simulink model "Model_31_02_2"  (R2024b)
settings: Solver=FixedStepAuto  StartTime=0.0  StopTime=20  FixedStep=0.01  RelTol=1e-3
values from neighbouring files (symbols this model uses):
  b = pend1.b    [InversePODE.m]    (also in Laboratorio_2_Pendolo_inverso_struct.m = 0.001; TESTTT.m = 13.516; errori.m = 0.001; state_space1.m)
  c = pend1.c    [InversePODE.m]    (also in Laboratorio_2_Pendolo_inverso_struct.m = 0.1; TESTTT.m = 0.1; errori.m = 0.1; state_space1.m)
  F = -pend1.Kp*x_n_l_NL(:,3) - pend1.Kd * x_n_l_NL(:,4)    [Laboratorio_2_Pendolo_inverso_struct.m]    (also in TESTTT.m = -Kp*x_n_l_NL(:,3) - Kd * x_n_l_NL(:,4))
  g = pend1.g    [InversePODE.m]    (also in InversePODE_RNL.m; Laboratorio_2_Pendolo_inverso_struct.m = 9.81; TESTTT.m = 9.81; errori.m = 9.81)
  l = pend1.l    [InversePODE.m]    (also in InversePODE_RNL.m; Laboratorio_2_Pendolo_inverso_struct.m = 0.75; TESTTT.m = 0.75; errori.m = 0.75)
  M = pend1.M    [InversePODE.m]    (also in InversePODE_RNL.m; Laboratorio_2_Pendolo_inverso_struct.m = 3; TESTTT.m = 3; errori.m = 3)
  m = pend1.m    [InversePODE.m]    (also in InversePODE_RNL.m; Laboratorio_2_Pendolo_inverso_struct.m = 0.1; TESTTT.m = 0.1; errori.m = 0.1)
  x0 = [0; 0; pi; 0]    [Laboratorio_2_Pendolo_inverso_struct.m]    (also in TESTTT.m = [0;0;0;0]; errori.m)
settings Model: Creator=baron  LastModifiedBy=baron

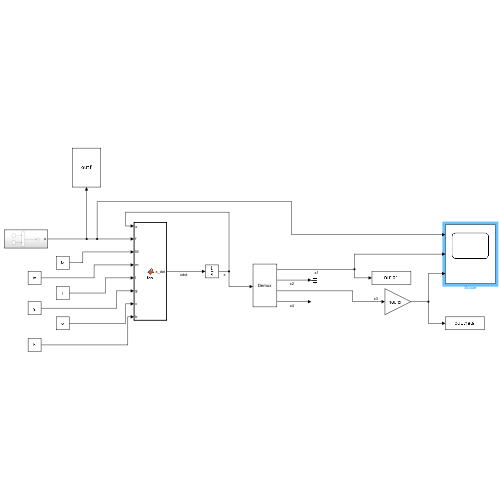
[thumbnail: Simulink's stored preview of the top-level diagram]
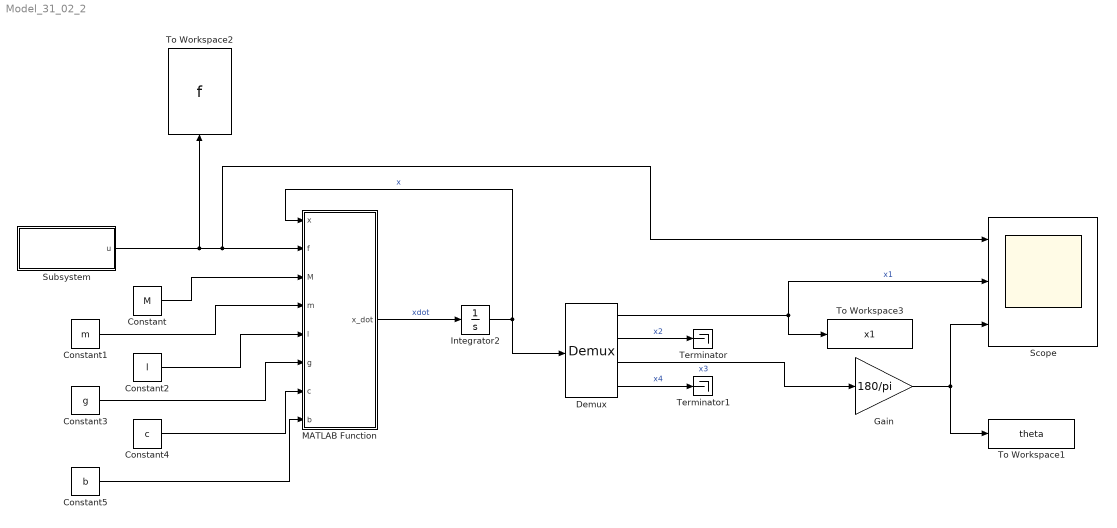
== system Model_31_02_2 ==
  Constant : Constant  Value=M
  Constant1 : Constant  Value=m
  Constant2 : Constant  Value=l
  Constant3 : Constant  Value=g
  Constant4 : Constant  Value=c
  Constant5 : Constant  Value=b
  Demux : Demux
      settings: DisplayOption=none
  Gain : Gain  Gain=180/pi
  Integrator2 : Integrator  InitialCondition=x0
  MATLAB Function : MATLAB Function  TreatAsAtomicUnit=on
  Scope : Scope  NumInputPorts=3
  Subsystem : Subsystem
  Terminator : Terminator
  Terminator1 : Terminator
  To Workspace1 : ToWorkspace  VariableName=theta  SampleTime=-1
      settings: Save2DSignal=2-D array (concatenate along first dimension)
  To Workspace2 : ToWorkspace  VariableName=f  SampleTime=-1
      settings: Save2DSignal=2-D array (concatenate along first dimension)
  To Workspace3 : ToWorkspace  VariableName=x1  SampleTime=-1
      settings: Save2DSignal=2-D array (concatenate along first dimension)
  wires:
  Constant3/1 -> MATLAB Function/6(g)
  Demux/2 -> Terminator/1  "x2"
  Constant1/1 -> MATLAB Function/4(m)
  Subsystem/1(u) -> Scope/1, MATLAB Function/2(f), To Workspace2/1
  Demux/1 -> Scope/2, To Workspace3/1  "x1"
  Constant/1 -> MATLAB Function/3(M)
  Integrator2/1 -> Demux/1, MATLAB Function/1(x)  "x"
  MATLAB Function/1(x_dot) -> Integrator2/1  "xdot"
  Constant2/1 -> MATLAB Function/5(l)
  Constant4/1 -> MATLAB Function/7(c)
  Constant5/1 -> MATLAB Function/8(b)
  Demux/4 -> Terminator1/1  "x4"
  Demux/3 -> Gain/1  "x3"
  Gain/1 -> To Workspace1/1, Scope/3

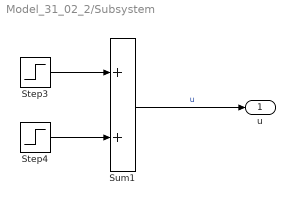
== system Model_31_02_2/Subsystem ==
  Step3 : Step  After=F  SampleTime=0
  Step4 : Step  Time=2  After=-F  SampleTime=0
  Sum1 : Sum
  u : Outport
  wires:
  Sum1/1 -> u/1  "u"
  Step4/1 -> Sum1/2
  Step3/1 -> Sum1/1

== matlab function Model_31_02_2/MATLAB Function ==
  data: x input; f input; x_dot output; M input; m input; l input; g input; c input; b input
function x_dot = fcn(x, f, M, m, l, g, c, b)

x1 = x(1);
x2 = x(2);
x3 = x(3);
x4 = x(4);

xdot1 = x2;
xdot2 = ((b/l)*x4*cos(x3) + m*g*sin(x3)*cos(x3) + m*l*(x4^2)*sin(x3) -c*x2 +f)/(M+m-m*cos(x3));
xdot3 = x4;
xdot4 = ((-m)/(M+m)*(x4^2)*cos(x3)*sin(x3) +c/((M+m)*l)*x2*cos(x3) - f/((M+m)*l)*cos(x3) -b/(m*l^2)*x4 +g/l*sin(x3))/(1-m/(M+m)*(cos(x3)^2));

x_dot = [xdot1; xdot2; xdot3; xdot4];
